simulink model "fuelcell"  (R2024b)
settings: Solver=ode23tb  StartTime=0.0  StopTime=0.001  RelTol=1e-3
undefined symbols (not defined in the file): DiscIntNeverNeededParam
libraries: spsSeriesRLCBranchLib x3, spsVoltageMeasurementLib x3, spsCurrentMeasurementLib x2, simulink x2, spsControlledCurrentSourceLib x1, spsControlledVoltageSourceLib x1, spsEdgeDetectorLib x1, spsSampleandHoldLib x1, spsFuelCellStackLib x1, spspowerguiLib x1
settings Model: Creator=LOUZAZNI  LastModifiedBy=Mahesh
settings SolverCC: AlgebraicLoopSolver=TrustRegion
settings DebuggingCC: UnconnectedInputMsg=warning  UnconnectedOutputMsg=warning  UnconnectedLineMsg=warning
settings ModelReferenceCC: EnableRefExpFcnMdlSchedulingChecks=on
settings SFSimCC: CustomCodeUndefinedFunction=UseInterfaceOnly
settings RTWCC: GPUComputeCapability=3.5

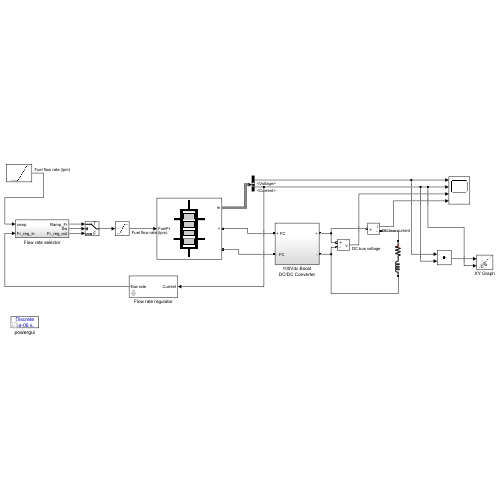
[thumbnail: Simulink's stored preview of the top-level diagram]
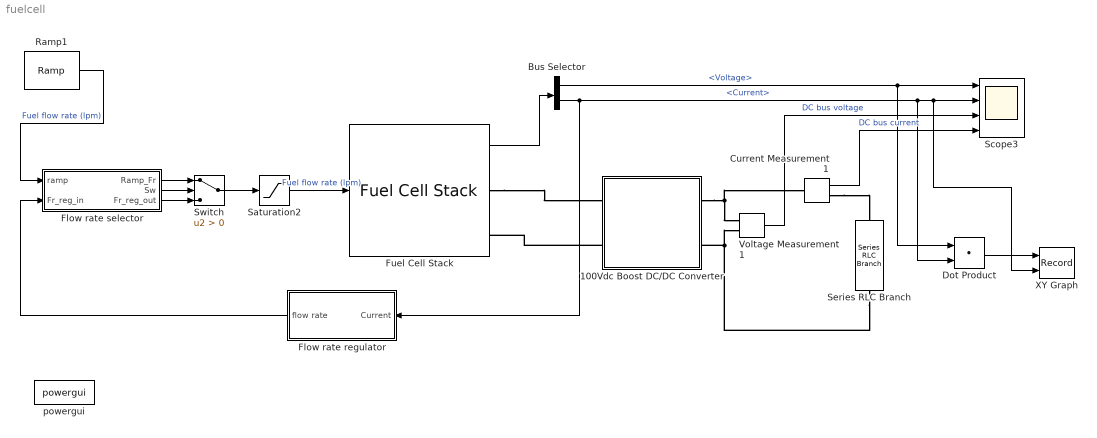
== system fuelcell ==
  100Vdc Boost DC/DC Converter : Subsystem
  Bus Selector : BusSelector  OutputSignals=Voltage,Current
  Current Measurement1 : spsCurrentMeasurementLib/Current Measurement  PhasorSimulation=off  OutputType=Complex  PSBequivalent=0
  Dot Product : DotProduct  OutDataTypeStr=Inherit: Inherit via internal rule
  Flow rate regulator : Subsystem  mask{Nc=65, Uf_H2=99.56, T=65, Pf=1.5, x=99.95}
      mask prompts: Nc "Number of cells"; Uf_H2 "Nominal Hydrogen utilization (%)"; T "Operating temperature (Celsius)"; Pf "Fuel pressure (bar)"; x "H2 composition (%)"
  Flow rate selector : Subsystem
  Fuel Cell Stack : spsFuelCellStackLib/Fuel Cell Stack  PresetModel=PEMFC - 6 kW - 45 Vdc  FcType=Proton Exchange Membrane (PEM)  Detailed=Detailed  Eoc=[65,63]  NomVI=[133.3,45]  EndVI=[225,37]  Nc=65  n=55  TOp=65  AirFr=300  SuppPress=[1.5,1]  Comp=[99.95,21,1]  SignX=off  SignY=off  FlowRateH2=on  FlowRateAir=off  SystemTemp=off  SystemPH2=off  SystemPAir=off  FCDyn=off  FC_tau=0  Peak_O2=80  V_Under=10
  Ramp1 : simulink/Sources/Ramp  slope=10  start=10  InitialOutput=0
  Saturation2 : Saturate  UpperLimit=85  LowerLimit=0
  Scope3 : Scope  NumInputPorts=4
  Series RLC Branch : spsSeriesRLCBranchLib/Series RLC Branch  LConnTagsString=__new0  RConnTagsString=__new0  BranchType=RL  Resistance=100*100/6000  Inductance=100*100/6000  SetiL0=off  InitialCurrent=0  Capacitance=1e-6  Setx0=off  InitialVoltage=0  Measurements=None
  Switch : Switch  Criteria=u2 > Threshold  SaturateOnIntegerOverflow=off  InputSameDT=off
  Voltage Measurement1 : spsVoltageMeasurementLib/Voltage Measurement  PhasorSimulation=off  OutputType=Complex  PSBequivalent=0
  XY Graph : Record  FileSettingsInternal="{\"entries\":[{\"content\":{\"excelSettings\":{\"content\":{},\"type\":\"Streamout.ExcelSettings\"}},\"type\":\"Streamout.FileSettingStorage\",\"uuid\":\"\"}],\"packageUris\":[\"http:\\/\\/schema.mathworks.com\\/mf0\\/streamout_blocks\\/R2020a\"],\"version\":\"1.0\"}"  Layout=[1 1]  SignalsInternal="{\"entries\":[{\"content\":{\"signals\":[{\"content\":{\"blockPath\":[],\"dimensions\":[1],\"domain\":\"\",\"lineColor\":\"#a2142f\",\"plots\":[ 1 ],\"port\":1,\"sid\":[\"\"],\"signalID\":1,\"signalName\":\"Dot Product\"},\"type\":\"RecordBlkView.Signal\",\"uuid\":\"\"},{\"content\":{\"blockPath\":[],\"dimensions\":[1],\"domain\":\"\",\"lineColor\":\"#139fff\",\"plots\":[ 1 ],\"port\":2,\"sid\":[\"\"],\"signalID\":2,\"signalName\":\"<Current>\"},\"type\":\"RecordBlkView.Signal\",\"uuid\":\"\"}]},\"type\":\"RecordBlkView.InputSignals\",\"uuid\":\"\"}],\"packageUris\":[\"http:\\/\\/schema.mathworks.com\\/mf0\\/streamout_blocks\\/R2020a\"],\"version\":\"1.0\"}"  VisualizationBindings="{\"xyplotplugin\":{\"info\":[{\"series\":[{\"bindingParametersList\":[{\"parameter\":\"X-Axis\",\"signalID\":2,\"signalName\":\"<Current>\"},{\"parameter\":\"Y-Axis\",\"signalID\":1,\"signalName\":\"Dot Product\"}],\"seriesID\":0}],\"subplotID\":1}]}}"  CompatibilityTag=XY
  powergui : spspowerguiLib/powergui  SimulationMode=Discrete  SampleTime=1e-6  frequency=60  Iterations=50  frequencyindice=0  Pbase=100e6  ErrMax=1e-4  UnitsV=kV  UnitsW=MW  buscounter=0  FunctionMessages=off  echomessages=off  EnableUseOfTLC=off  CurrentSourceSwitches=off  DisableSnubberDevices=off  DisableRonSwitches=off  DisableVfSwitches=off  DisplayEquations=off  AutomaticDiscreteSolvers=off  SolverType=Tustin  Interpol=off  ExternalGateDelay=off  methode=off  Ts=0  x0status=blocks  SPID=off  SwTol=0  HookPort=off  NonlinearTolerance=0  nMaxIteration=15  ContinueOnMaxIteration=off  RestoreLinks=warning  ResistiveCurrentMeasurement=off  Frange=[0:2:500]  Ylog=off  Xlog=on  ShowGrid=off  save=off  variable=ZData  structure=ScopeData1  ZoomFFT=off  StartTime=0.0  cycles=1  DisplayStyle=1  fundamental=60  FreqAxis=on  MaxFrequency=1000  frequencyindicesteady=1  RmsSteady=1  display=off
  wires:
  Flow rate selector/3(Fr_reg_out) -> Switch/3
  Saturation2/1 -> Fuel Cell Stack/1  "Fuel flow rate (lpm)"
  Ramp1/1 -> Flow rate selector/1(ramp)  "Fuel flow rate (lpm)"
  Voltage Measurement1/1 -> Scope3/3  "DC bus voltage"
  Flow rate regulator/1(flow rate) -> Flow rate selector/2(Fr_reg_in)
  Bus Selector/1 -> Dot Product/1, Scope3/1  "<Voltage>"
  Flow rate selector/2(Sw) -> Switch/2
  Current Measurement1/1 -> Scope3/4  "DC bus current"
  Flow rate selector/1(Ramp_Fr) -> Switch/1
  Bus Selector/2 -> Dot Product/2, XY Graph/2, Scope3/2, Flow rate regulator/1(Current)  "<Current>"
  Fuel Cell Stack/1 -> Bus Selector/1
  Switch/1 -> Saturation2/1
  Dot Product/1 -> XY Graph/1
  connections:
  Current Measurement1/RConn1 -- Series RLC Branch/LConn1
  Series RLC Branch/RConn1 -- Voltage Measurement1/LConn2 -- 100Vdc Boost DC/DC Converter/RConn2
  100Vdc Boost DC/DC Converter/RConn1 -- Voltage Measurement1/LConn1 -- Current Measurement1/LConn1
  100Vdc Boost DC/DC Converter/LConn2 -- Fuel Cell Stack/RConn2
  Fuel Cell Stack/RConn1 -- 100Vdc Boost DC/DC Converter/LConn1

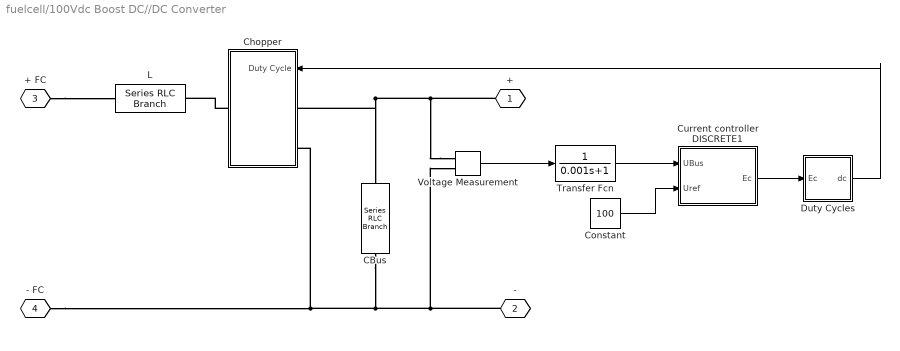
== system fuelcell/100Vdc Boost DC//DC Converter ==
  CBus : spsSeriesRLCBranchLib/Series RLC Branch  LConnTagsString=__new0  RConnTagsString=__new0  BranchType=RC  Resistance=0.2  Inductance=1e-3  SetiL0=off  InitialCurrent=0  Capacitance=7500e-6  Setx0=on  InitialVoltage=100  Measurements=None
  Chopper : Subsystem  mask(SPSdrives Converter){SnubberResistance=10e3, SnubberCapacitance=inf, Ron=1e-3, ForwardVoltages=[1.3,1.3], IGBTParameters=[0,0], converterType=Inverter}
      mask prompts: SnubberResistance "Snubber resistance Rs (Ohms):"; SnubberCapacitance "Snubber capacitance Cs (F):"; Ron "Ron (Ohms):"; ForwardVoltages "Forward voltages [Device Vf(V), Diode Vd (V)]"; IGBTParameters "[Tf(s), Tt(s)]:"; converterType "Converter type:"
      mask help: This model implements an average-value buck converter."Duty Cycle" contains the duty cycle of the internal IGBT device.
      mask TypeOptions converterType: Rectifier | Inverter
      mask Display: plot(0,0,100,100,[39 39 23.8],[71 28 28],[44 56 49.6 56 52.8 56 61 61],[39.2 33.6 32.8 33.6 40.8 33.6 30 12.4],[44 44 44 61 61],[28 71 60 66.4 90],[75 67 83 75 67 83 75 75],[54 42 42 54 54 54 54 66],[61 75 75],[24 24 42],[75 75 61],[66,76,76])
  Constant : Constant  Value=100
  Current controller DISCRETE1 : Subsystem  mask(PI controller){Kp=0.0005, Ki=0.15, Ts=1e-3}
      mask prompts: Kp "Proportional gain (Kp)"; Ki "Integral gain (Ki)"; Ts "Sample time (s) :"
      mask help: Proportional-Integral Speed Controller
      mask Display: plot(0,0,100,100,[35,35,65],[70,30,30],[35,65],[45,60])
  Duty Cycles : Subsystem
  L : spsSeriesRLCBranchLib/Series RLC Branch  LConnTagsString=__new0  RConnTagsString=__new0  BranchType=L  Resistance=0.3  Inductance=500e-6  SetiL0=off  InitialCurrent=0  Capacitance=100e-6  Setx0=off  InitialVoltage=0  Measurements=None
  Transfer Fcn : TransferFcn  Denominator=[0.001 1]
  Voltage Measurement : spsVoltageMeasurementLib/Voltage Measurement  PhasorSimulation=off  OutputType=Complex  PSBequivalent=0
  + : PMIOPort  Tag=PMCPort  Side=Right
  - : PMIOPort  Tag=PMCPort  Port=2  Side=Right
  + FC : PMIOPort  Tag=PMCPort  Port=3  Side=Left
  - FC : PMIOPort  Tag=PMCPort  Port=4  Side=Left
  wires:
  Constant/1 -> Current controller DISCRETE1/2(Uref)
  Voltage Measurement/1 -> Transfer Fcn/1
  Duty Cycles/1(dc) -> Chopper/1(Duty Cycle)
  Transfer Fcn/1 -> Current controller DISCRETE1/1(UBus)
  Current controller DISCRETE1/1(Ec) -> Duty Cycles/1(Ec)
  connections:
  - FC/RConn1 -- Voltage Measurement/LConn2 -- -/RConn1 -- CBus/RConn1 -- Chopper/LConn2
  Voltage Measurement/LConn1 -- +/RConn1 -- Chopper/LConn1 -- CBus/LConn1
  Chopper/RConn1 -- L/LConn1
  + FC/RConn1 -- L/RConn1

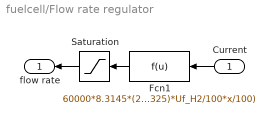
== system fuelcell/Flow rate regulator ==
  Current : Inport
  Fcn1 : Fcn  Expr=60000*8.3145*(273+T)*Nc*u(1)/(2*96485*(Pf*101325)*Uf_H2/100*x/100)
  Saturation : Saturate  UpperLimit=inf  LowerLimit=1
  flow rate : Outport  VectorParamsAs1DForOutWhenUnconnected=off
  wires:
  Fcn1/1 -> Saturation/1
  Current/1 -> Fcn1/1
  Saturation/1 -> flow rate/1

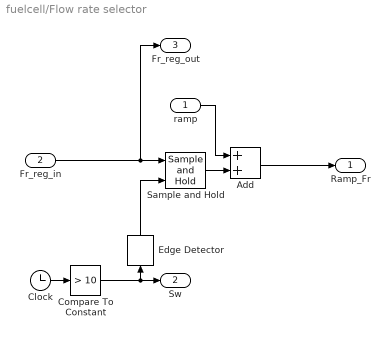
== system fuelcell/Flow rate selector ==
  ramp : Inport
  Fr_reg_in : Inport  Port=2
  Add : Sum
  Clock : Clock
  Compare To Constant : simulink/Logic and Bit Operations/Compare To Constant  relop=>  const=10  OutDataTypeStr=boolean
  Edge Detector : spsEdgeDetectorLib/Edge Detector  model=Rising  ic=0  Ts=0
  Sample and Hold : spsSampleandHoldLib/Sample and Hold  ic=0  Ts=0
  Ramp_Fr : Outport  VectorParamsAs1DForOutWhenUnconnected=off
  Sw : Outport  Port=2  VectorParamsAs1DForOutWhenUnconnected=off
  Fr_reg_out : Outport  Port=3  VectorParamsAs1DForOutWhenUnconnected=off
  wires:
  Clock/1 -> Compare To Constant/1
  Compare To Constant/1 -> Edge Detector/1, Sw/1
  Edge Detector/1 -> Sample and Hold/2
  Sample and Hold/1 -> Add/2
  Fr_reg_in/1 -> Sample and Hold/1, Fr_reg_out/1
  ramp/1 -> Add/1
  Add/1 -> Ramp_Fr/1

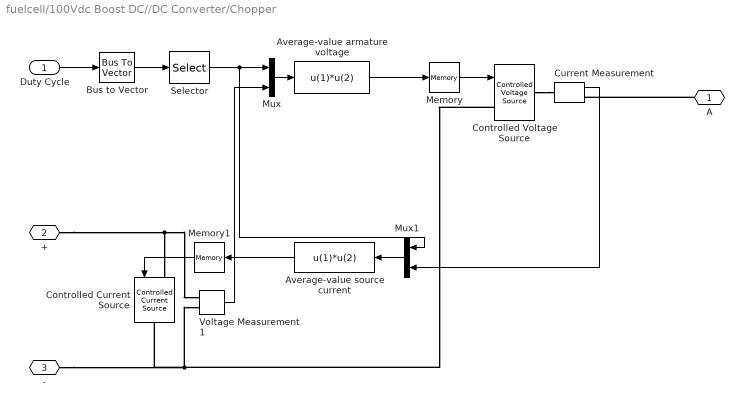
== system fuelcell/100Vdc Boost DC//DC Converter/Chopper ==
  Duty Cycle : Inport
  Average-value armature voltage : Fcn  Expr=u(1)*u(2)
  Average-value source current : Fcn  Expr=u(1)*u(2)
  Bus to Vector : BusToVector
  Controlled Current Source : spsControlledCurrentSourceLib/Controlled Current Source  Initialize=on  Source_Type=AC  Amplitude=0  Phase=0  Frequency=0  Measurements=None
  Controlled Voltage Source : spsControlledVoltageSourceLib/Controlled Voltage Source  Initialize=on  Source_Type=AC  Amplitude=0  Phase=0  Frequency=0  Measurements=None
  Current Measurement : spsCurrentMeasurementLib/Current Measurement  Tag=PoWeRsYsTeMmEaSuReMeNt  PhasorSimulation=off  OutputType=Magnitude  PSBequivalent=0
      settings: AttributesFormatString=\n
  Memory : Memory
  Memory1 : Memory
  Mux : Mux  Inputs=2
  Mux1 : Mux  Inputs=2
  Selector : Selector  InputPortWidth=2  IndexOptions=Index vector (dialog)  Indices=[1]  OutputSizes=1
  Voltage Measurement1 : spsVoltageMeasurementLib/Voltage Measurement  Tag=PoWeRsYsTeMmEaSuReMeNt  PhasorSimulation=off  OutputType=Magnitude  PSBequivalent=0
  A : PMIOPort  Side=Right
  + : PMIOPort  Port=2  Side=Left
  - : PMIOPort  Port=3  Side=Left
  wires:
  Selector/1 -> Mux1/1, Mux/1
  Memory1/1 -> Controlled Current Source/1
  Average-value source current/1 -> Memory1/1
  Current Measurement/1 -> Mux1/2
  Mux1/1 -> Average-value source current/1
  Duty Cycle/1 -> Bus to Vector/1
  Voltage Measurement1/1 -> Mux/2
  Mux/1 -> Average-value armature voltage/1
  Average-value armature voltage/1 -> Memory/1
  Memory/1 -> Controlled Voltage Source/1
  Bus to Vector/1 -> Selector/1
  connections:
  A/RConn1 -- Current Measurement/RConn1
  Controlled Voltage Source/RConn1 -- Current Measurement/LConn1
  +/RConn1 -- Voltage Measurement1/LConn1 -- Controlled Current Source/LConn1
  Controlled Voltage Source/LConn1 -- -/RConn1 -- Controlled Current Source/RConn1 -- Voltage Measurement1/LConn2

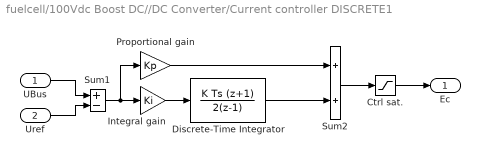
== system fuelcell/100Vdc Boost DC//DC Converter/Current controller DISCRETE1 ==
  UBus : Inport
  Uref : Inport  Port=2
  Ctrl sat. : Saturate  UpperLimit=0.95  LowerLimit=-0.95
  Discrete-Time Integrator : DiscreteIntegrator  IntegratorMethod=Integration: Trapezoidal  SampleTime=Ts  LimitOutput=on  UpperSaturationLimit=0.95  LowerSaturationLimit=-0.95  ICPrevOutput=DiscIntNeverNeededParam  ICPrevScaledInput=DiscIntNeverNeededParam
  Integral gain : Gain  Gain=Ki  SaturateOnIntegerOverflow=on  OutDataTypeStr=Inherit: Same as input  ParamDataTypeStr=Inherit: Same as input
  Proportional gain : Gain  Gain=Kp  SaturateOnIntegerOverflow=on  OutDataTypeStr=Inherit: Same as input  ParamDataTypeStr=Inherit: Same as input
  Sum1 : Sum  Inputs=+-  InputSameDT=on  SaturateOnIntegerOverflow=on  OutDataTypeStr=Inherit: Same as first input
  Sum2 : Sum  InputSameDT=on  SaturateOnIntegerOverflow=on  OutDataTypeStr=Inherit: Same as first input
  Ec : Outport  InitialOutput=0  VectorParamsAs1DForOutWhenUnconnected=off
  wires:
  Ctrl sat./1 -> Ec/1
  Sum2/1 -> Ctrl sat./1
  Discrete-Time Integrator/1 -> Sum2/2
  Uref/1 -> Sum1/2
  UBus/1 -> Sum1/1
  Sum1/1 -> Proportional gain/1, Integral gain/1
  Integral gain/1 -> Discrete-Time Integrator/1
  Proportional gain/1 -> Sum2/1

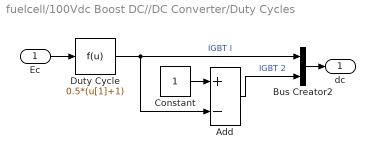
== system fuelcell/100Vdc Boost DC//DC Converter/Duty Cycles ==
  Ec : Inport
  Add : Sum  Inputs=+-
  Bus Creator2 : BusCreator  Inputs=2
  Constant : Constant
  Duty Cycle : Fcn  Expr=0.5*(u[1]+1)
  dc : Outport  VectorParamsAs1DForOutWhenUnconnected=off
  wires:
  Bus Creator2/1 -> dc/1
  Ec/1 -> Duty Cycle/1
  Constant/1 -> Add/1
  Add/1 -> Bus Creator2/2  "IGBT 2"
  Duty Cycle/1 -> Bus Creator2/1, Add/2  "IGBT I"
